simulink model "SensorProcessing_session_for_integrated"  (R2025b)
settings: Solver=FixedStepDiscrete  StartTime=0.0  StopTime=10.0  FixedStep=0.1  RelTol=1e-3
settings Model: Creator=Ahmed  LastModifiedBy=LENOVO

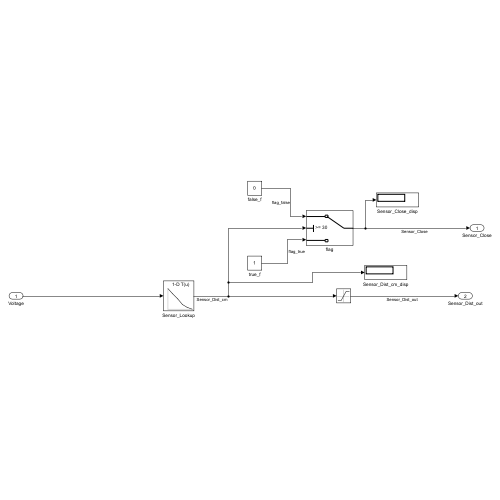
[thumbnail: Simulink's stored preview of the top-level diagram]
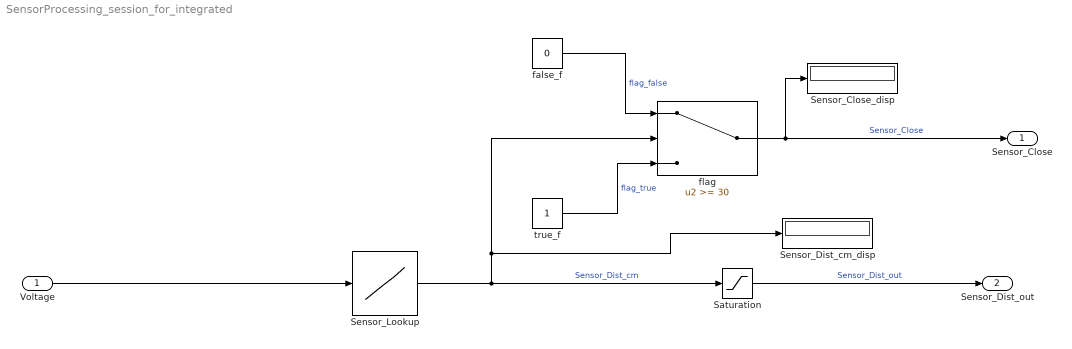
== system SensorProcessing_session_for_integrated ==
  Voltage : Inport  OutDataTypeStr=double
  Saturation : Saturate  UpperLimit=400  LowerLimit=0
  Sensor_Close_disp : Display
  Sensor_Dist_cm_disp : Display
  Sensor_Lookup : Lookup_n-D  NumberOfTableDimensions=1  BreakpointsForDimension1=[0 1 2 3 4 5]  Table=[400 300 200 100 50 10]  ExtrapMethod=Clip  InternalRulePriority=Speed  RndMeth=Simplest
  false_f : Constant  Value=0
  flag : Switch  Threshold=30  SaturateOnIntegerOverflow=off  InputSameDT=off
  true_f : Constant  OutDataTypeStr=Inherit: Inherit via back propagation
  Sensor_Close : Outport  OutDataTypeStr=boolean
  Sensor_Dist_out : Outport  Port=2  OutDataTypeStr=double
  wires:
  Voltage/1 -> Sensor_Lookup/1
  false_f/1 -> flag/1  "flag_false"
  flag/1 -> Sensor_Close/1, Sensor_Close_disp/1  "Sensor_Close"
  Sensor_Lookup/1 -> Sensor_Dist_cm_disp/1, flag/2, Saturation/1  "Sensor_Dist_cm"
  true_f/1 -> flag/3  "flag_true"
  Saturation/1 -> Sensor_Dist_out/1  "Sensor_Dist_out"
